simulink library "planetary_gear_lib"  (R2025a)
settings: Solver=VariableStepAuto  StartTime=0.0  StopTime=10.0  RelTol=1e-3
undefined symbols (not defined in the file): cvtPar, Local, rad_planet, rad_sun, X, Y, Z
libraries: sm_lib x24, Multibody_Parts_Lib x15, nesl_utility x2
Description:
  | Copyright 2023-2025 The MathWorks, Inc.
settings Model: Creator=smiller  LastModifiedBy=smiller
settings RTWCC: GPUComputeCapability=3.5

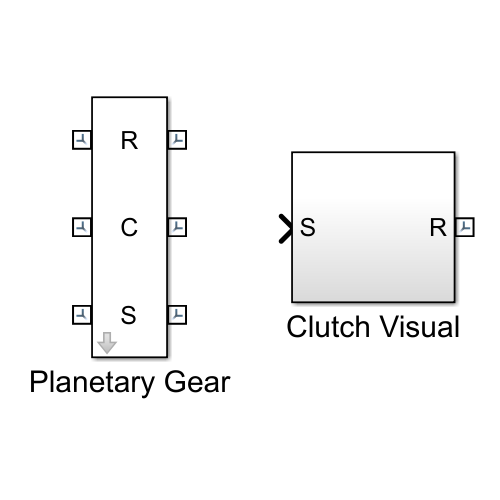
[thumbnail: Simulink's stored preview of the top-level diagram]
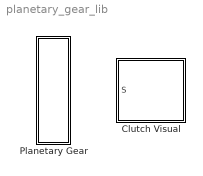
== system planetary_gear_lib ==
  Clutch Visual : Subsystem
  Planetary Gear : Subsystem  Tag=PublishSubsystem  mask{rad_sun=0.78, nteeth_sun=45, rad_planet=0.26, nteeth_planet=15, rad_ring=2*rad_planet+rad_sun, nteeth_ring=75, pg_axial_offset=2, gear_thickness=cvtPar.gear_thickness, link_thickness=cvtPar.link_thickness, rad_hole=cvtPar.rad_hole, ring_gear_clr=[0.0 0.4 0.6], sun_gear_clr=[0.8 0.8 0.3], pla_gear_clr=[0.8 0.8 0.8], carrier_color=[0.5 0.5 0.5]}
      mask prompts: rad_sun "Sun Pitch Radius"; nteeth_sun "Sun # Teeth"; rad_planet "Planet Pitch Radius"; nteeth_planet "Planet # Teeth"; rad_ring "Ring Pitch Radius"; nteeth_ring "Ring # Teeth"; pg_axial_offset "Offset to Planetary Gear (m)"; gear_thickness "Gear Thickness (m)"; link_thickness "Link Thickness (m)"; rad_hole "Gear Hole Radius (m)"; ring_gear_clr "Ring Gear Color [RGB]"; sun_gear_clr "Sun Gear Color [RGB]"; pla_gear_clr "Planet Gear Color [RGB]"; carrier_color "Carrier Color [RGB]"
      mask TypeOptions ring_gear_clr:
      | Ring
      | Gear/gear_clr
      mask TypeOptions sun_gear_clr:
      | Sun
      | Gear/gear_clr
      mask TypeOptions pla_gear_clr: Planet 1/gear_clr | Planet 2/gear_clr | Planet 3/gear_clr
      mask TypeOptions carrier_color:
      | Carrier
      | Gear/carrier_color

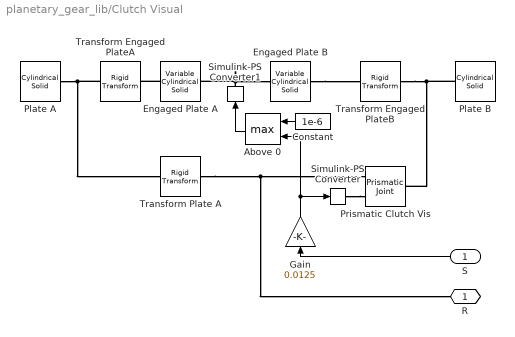
== system planetary_gear_lib/Clutch Visual ==
  S : Inport
  Above 0 : MinMax  Function=max  Inputs=2  ZeroCross=off
  Constant : Constant  Value=1e-6
  Engaged Plate A : sm_lib/Body Elements/Variable Mass/Variable Cylindrical Solid  RadiusType=Constant  Radius=0.025*2+0.001  RadiusUnits=m  LengthType=ProvidedByInput  Length=1  LengthUnits=m  MassType=CalculateFromGeometry  Density=1  DensityUnits=kg/m^3  SenseRadius=off  SenseLength=off  SenseMass=off  SenseCenterOfMass=off  SenseInertiaMatrix=off  GraphicType=FromGeometry  MarkerShape=Sphere  MarkerSize=10  GraphicVisPropType=SimpleVisualProperties  GraphicDiffuseColor=[0.902 0.4784 0.4784]  GraphicOpacity=1.0  GraphicSpecularColor=[0.5 0.5 0.5 1.0]  GraphicAmbientColor=[0.15 0.15 0.15 1.0]  GraphicEmissiveColor=[0.0 0.0 0.0 1.0]  GraphicShininess=75
  Engaged Plate B : sm_lib/Body Elements/Variable Mass/Variable Cylindrical Solid  RadiusType=Constant  Radius=0.025*2+0.001  RadiusUnits=m  LengthType=ProvidedByInput  Length=1  LengthUnits=m  MassType=CalculateFromGeometry  Density=1  DensityUnits=kg/m^3  SenseRadius=off  SenseLength=off  SenseMass=off  SenseCenterOfMass=off  SenseInertiaMatrix=off  GraphicType=FromGeometry  MarkerShape=Sphere  MarkerSize=10  GraphicVisPropType=SimpleVisualProperties  GraphicDiffuseColor=[1 0 0]  GraphicOpacity=1.0  GraphicSpecularColor=[0.5 0.5 0.5 1.0]  GraphicAmbientColor=[0.15 0.15 0.15 1.0]  GraphicEmissiveColor=[0.0 0.0 0.0 1.0]  GraphicShininess=75
  Gain : Gain  Gain=0.0125
  Plate A : sm_lib/Body Elements/Cylindrical Solid  CylinderRadius=0.025*2  CylinderRadiusUnits=m  CylinderLength=0.0125-0.0001  CylinderLengthUnits=m  ExportEntireGeometry=off  InertiaType=CalculateFromGeometry  BasedOnType=Density  Density=1000  DensityUnits=kg/m^3  Mass=1  MassUnits=kg  CenterOfMass=[0 0 0]  CenterOfMassUnits=m  MomentsOfInertia=[1 1 1]  MomentsOfInertiaUnits=kg*m^2  ProductsOfInertia=[0 0 0]  ProductsOfInertiaUnits=kg*m^2  GraphicType=FromGeometry  MarkerShape=Sphere  MarkerSize=10  GraphicVisPropType=SimpleVisualProperties  GraphicDiffuseColor=[1.0 1.0 1.0]  GraphicOpacity=1.0  GraphicSpecularColor=[0.5 0.5 0.5 1.0]  GraphicAmbientColor=[0.15 0.15 0.15 1.0]  GraphicEmissiveColor=[0.0 0.0 0.0 1.0]  GraphicShininess=75  DoExposeReferenceFrame=off  SerializedFrames=<Frames><Frame><Id>Frame1</Id><Value><Name>B</Name><Origin><Source>GeometricFeature</Source><FeatureName>bottom surface</FeatureName></Origin><PrimaryAxis><DefinedDirection>+Z</DefinedDirection><Source>ReferenceFrame</Source><SourceDirection>+Z</SourceDirection><FeatureName></FeatureName></PrimaryAxis><SecondaryAxis><DefinedDirection>+X</DefinedDirection><Source>ReferenceFrame</Source><SourceDirection>+X</SourceDirection><FeatureName></FeatureName></SecondaryAxis></Value></Frame></Frames>
  Plate B : sm_lib/Body Elements/Cylindrical Solid  CylinderRadius=0.025*2  CylinderRadiusUnits=m  CylinderLength=0.0125-0.0001  CylinderLengthUnits=m  ExportEntireGeometry=off  InertiaType=CalculateFromGeometry  BasedOnType=Density  Density=1000  DensityUnits=kg/m^3  Mass=1  MassUnits=kg  CenterOfMass=[0 0 0]  CenterOfMassUnits=m  MomentsOfInertia=[1 1 1]  MomentsOfInertiaUnits=kg*m^2  ProductsOfInertia=[0 0 0]  ProductsOfInertiaUnits=kg*m^2  GraphicType=FromGeometry  MarkerShape=Sphere  MarkerSize=10  GraphicVisPropType=SimpleVisualProperties  GraphicDiffuseColor=[1.0 1.0 1.0]  GraphicOpacity=1.0  GraphicSpecularColor=[0.5 0.5 0.5 1.0]  GraphicAmbientColor=[0.15 0.15 0.15 1.0]  GraphicEmissiveColor=[0.0 0.0 0.0 1.0]  GraphicShininess=75  DoExposeReferenceFrame=off  SerializedFrames=<Frames><Frame><Id>Frame1</Id><Value><Name>F</Name><Origin><Source>GeometricFeature</Source><FeatureName>top surface</FeatureName></Origin><PrimaryAxis><DefinedDirection>+Z</DefinedDirection><Source>ReferenceFrame</Source><SourceDirection>+Z</SourceDirection><FeatureName></FeatureName></PrimaryAxis><SecondaryAxis><DefinedDirection>+X</DefinedDirection><Source>ReferenceFrame</Source><SourceDirection>+X</SourceDirection><FeatureName></FeatureName></SecondaryAxis></Value></Frame></Frames>
  Prismatic Clutch Vis : sm_lib/Joints/Prismatic Joint  JointMode=Normal  CompositeWrenchDir=FollowerOnBase  CompositeWrenchFrame=BaseFrame  SenseConstraintForce=off  SenseConstraintTorque=off  SenseTotalForce=off  SenseTotalTorque=off  PositionTargetSpecify=off  PositionTargetPriority=High  PositionTargetValue=0  PositionTargetValueUnits=m  VelocityTargetSpecify=off  VelocityTargetPriority=High  VelocityTargetValue=0  VelocityTargetValueUnits=m/s  EquilibriumPosition=0  EquilibriumPositionUnits=m  SpringStiffness=0  SpringStiffnessUnits=N/m  DampingCoefficient=0  DampingCoefficientUnits=N/(m/s)  LowerLimitSpecify=off  LowerLimitBound=-1  LowerLimitBoundUnits=m  LowerLimitStiffness=1e6  LowerLimitStiffnessUnits=N/m  LowerLimitDamping=1e3  LowerLimitDampingUnits=N/(m/s)  LowerLimitTransitionRegionWidth=1e-4  LowerLimitTransitionRegionWidthUnits=m  UpperLimitSpecify=off  UpperLimitBound=1  UpperLimitBoundUnits=m  UpperLimitStiffness=1e6  UpperLimitStiffnessUnits=N/m  UpperLimitDamping=1e3  UpperLimitDampingUnits=N/(m/s)  UpperLimitTransitionRegionWidth=1e-4  UpperLimitTransitionRegionWidthUnits=m  TorqueActuationMode=ComputedTorque  MotionActuationMode=InputMotion  SensePosition=off  SenseVelocity=off  SenseAcceleration=off  SenseTorqueForce=off  SenseLowerLimitTorqueForce=off  SenseUpperLimitTorqueForce=off
  Simulink-PS Converter : nesl_utility/Simulink-PS Converter  PhysicalDomain=network_engine_domain  SubClassName=ps_input  LeftPortType=input  RightPortType=output  PseudoPeriodic=off  Frequencies=[]  NoiseDistribution=none  NoiseParameters=[]  Unit=1  AffineConversion=off  FilteringAndDerivatives=filter  SimscapeFilterOrder=2  InputFilterTimeConstant=0.001  UdotUserProvided=0
  Simulink-PS Converter1 : nesl_utility/Simulink-PS Converter  PhysicalDomain=network_engine_domain  SubClassName=ps_input  LeftPortType=input  RightPortType=output  PseudoPeriodic=off  Frequencies=[]  NoiseDistribution=none  NoiseParameters=[]  Unit=1  AffineConversion=off  FilteringAndDerivatives=filter  SimscapeFilterOrder=2  InputFilterTimeConstant=0.001  UdotUserProvided=0
  Transform Engaged PlateA : sm_lib/Frames and Transforms/Rigid Transform  RotationMethod=None  FollAlignAxisA=+X  BaseAlignAxisA=+Y  FollAlignAxisB=+Y  BaseAlignAxisB=+Z  RotationStandardAxis=+Z  RotationAngle=0.0  RotationAngleUnits=deg  RotationArbitraryAxis=[0 0 1]  RotationSequenceAxes=FollowerAxes  RotationSequence=XYX  RotationSequenceAngles=[0 0 0]  RotationSequenceAnglesUnits=deg  RotationMatrix=[1 0 0; 0 1 0; 0 0 1]  Quaternion=[1 0 0 0]  TranslationMethod=StandardAxis  TranslationCartesianOffset=[0 0 0]  TranslationCartesianOffsetUnits=m  TranslationStandardAxis=+Z  TranslationStandardOffset=1e-5  TranslationStandardOffsetUnits=m  TranslationROffset=0  TranslationROffsetUnits=m  TranslationThetaOffset=0  TranslationThetaOffsetUnits=deg  TranslationZOffset=0  TranslationZOffsetUnits=m
  Transform Engaged PlateB : sm_lib/Frames and Transforms/Rigid Transform  RotationMethod=StandardAxis  FollAlignAxisA=+X  BaseAlignAxisA=+Y  FollAlignAxisB=+Y  BaseAlignAxisB=+Z  RotationStandardAxis=+X  RotationAngle=180  RotationAngleUnits=deg  RotationArbitraryAxis=[0 0 1]  RotationSequenceAxes=FollowerAxes  RotationSequence=XYX  RotationSequenceAngles=[0 0 0]  RotationSequenceAnglesUnits=deg  RotationMatrix=[1 0 0; 0 1 0; 0 0 1]  Quaternion=[1 0 0 0]  TranslationMethod=StandardAxis  TranslationCartesianOffset=[0 0 0]  TranslationCartesianOffsetUnits=m  TranslationStandardAxis=+Z  TranslationStandardOffset=-1e-5  TranslationStandardOffsetUnits=m  TranslationROffset=0  TranslationROffsetUnits=m  TranslationThetaOffset=0  TranslationThetaOffsetUnits=deg  TranslationZOffset=0  TranslationZOffsetUnits=m
  Transform Plate A : sm_lib/Frames and Transforms/Rigid Transform  RotationMethod=None  FollAlignAxisA=+X  BaseAlignAxisA=+Y  FollAlignAxisB=+Y  BaseAlignAxisB=+Z  RotationStandardAxis=+Z  RotationAngle=0.0  RotationAngleUnits=deg  RotationArbitraryAxis=[0 0 1]  RotationSequenceAxes=FollowerAxes  RotationSequence=XYX  RotationSequenceAngles=[0 0 0]  RotationSequenceAnglesUnits=deg  RotationMatrix=[1 0 0; 0 1 0; 0 0 1]  Quaternion=[1 0 0 0]  TranslationMethod=StandardAxis  TranslationCartesianOffset=[0 0 0]  TranslationCartesianOffsetUnits=m  TranslationStandardAxis=+Z  TranslationStandardOffset=0.0125  TranslationStandardOffsetUnits=m  TranslationROffset=0  TranslationROffsetUnits=m  TranslationThetaOffset=0  TranslationThetaOffsetUnits=deg  TranslationZOffset=0  TranslationZOffsetUnits=m
  R : PMIOPort  Side=Right
  wires:
  Above 0/1 -> Simulink-PS Converter1/1
  Gain/1 -> Simulink-PS Converter/1, Above 0/2
  Constant/1 -> Above 0/1
  S/1 -> Gain/1
  connections:
  Transform Plate A/LConn1 -- Prismatic Clutch Vis/LConn1 -- R/RConn1
  Engaged Plate B/RConn1 -- Transform Engaged PlateB/LConn1
  Simulink-PS Converter1/RConn1 -- Engaged Plate A/LConn1 -- Engaged Plate B/LConn1
  Plate A/LConn1 -- Transform Engaged PlateA/LConn1 -- Transform Plate A/RConn1
  Transform Engaged PlateB/RConn1 -- Plate B/LConn1 -- Prismatic Clutch Vis/RConn1
  Simulink-PS Converter/RConn1 -- Prismatic Clutch Vis/LConn2
  Engaged Plate A/RConn1 -- Transform Engaged PlateA/RConn1

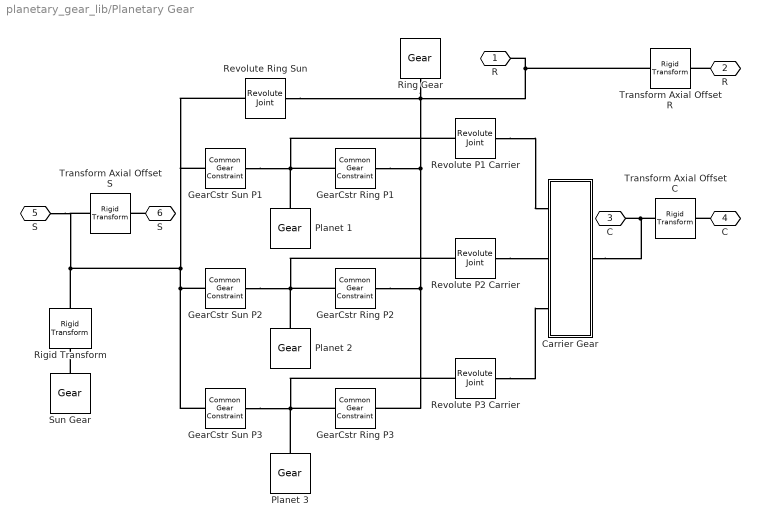
== system planetary_gear_lib/Planetary Gear ==
  Carrier Gear : Subsystem  Tag=PublishSubsystem  mask{carrier_color=carrier_color}
      mask prompts: carrier_color "Carrier Color [RGB]"
      mask TypeOptions carrier_color: Link End P1/circ_color | Link End P2/circ_color | Link End P3/circ_color | Link Seg P1/link_color | Link Seg P2/link_color | Link Seg P3/link_color | Rod P1/rod_color | Rod P2/rod_color | Rod P3/rod_color | Rod Sun/rod_color
  GearCstr Sun P1 : sm_lib/Gears and Couplings/Gears/Common Gear Constraint  GearType=External  SpecificationType=PitchCircleRadii  CenterDistance=20.0  CenterDistanceUnits=cm  GearRatio=1.0  BaseGearRadius=rad_sun  BaseGearRadiusUnits=m  FollGearRadius=rad_planet  FollGearRadiusUnits=m
  GearCstr Sun P2 : sm_lib/Gears and Couplings/Gears/Common Gear Constraint  GearType=External  SpecificationType=PitchCircleRadii  CenterDistance=20.0  CenterDistanceUnits=cm  GearRatio=1.0  BaseGearRadius=rad_sun  BaseGearRadiusUnits=m  FollGearRadius=rad_planet  FollGearRadiusUnits=m
  GearCstr Sun P3 : sm_lib/Gears and Couplings/Gears/Common Gear Constraint  GearType=External  SpecificationType=PitchCircleRadii  CenterDistance=20.0  CenterDistanceUnits=cm  GearRatio=1.0  BaseGearRadius=rad_sun  BaseGearRadiusUnits=m  FollGearRadius=rad_planet  FollGearRadiusUnits=m
  GearCstr Ring P1 : sm_lib/Gears and Couplings/Gears/Common Gear Constraint  GearType=Internal  SpecificationType=PitchCircleRadii  CenterDistance=20.0  CenterDistanceUnits=cm  GearRatio=1.0  BaseGearRadius=rad_ring  BaseGearRadiusUnits=m  FollGearRadius=rad_planet  FollGearRadiusUnits=m
  GearCstr Ring P2 : sm_lib/Gears and Couplings/Gears/Common Gear Constraint  GearType=Internal  SpecificationType=PitchCircleRadii  CenterDistance=20.0  CenterDistanceUnits=cm  GearRatio=1.0  BaseGearRadius=rad_ring  BaseGearRadiusUnits=m  FollGearRadius=rad_planet  FollGearRadiusUnits=m
  GearCstr Ring P3 : sm_lib/Gears and Couplings/Gears/Common Gear Constraint  GearType=Internal  SpecificationType=PitchCircleRadii  CenterDistance=20.0  CenterDistanceUnits=cm  GearRatio=1.0  BaseGearRadius=rad_ring  BaseGearRadiusUnits=m  FollGearRadius=rad_planet  FollGearRadiusUnits=m
  Planet 1 : Multibody_Parts_Lib/Gears/Gear  popup_gear_type=External  gear_pd=rad_planet*2  gear_nt=nteeth_planet  gear_th=gear_thickness  gear_rh=rad_hole  gear_rt=0.02  gear_rho=7000  gear_clr=pla_gear_clr  gear_opc=1  popup_ad_dd=Default  gear_ad=0.125/12  gear_dd=1.157*0.125/12  popup_markings=Two  mark_radius_range=[0.6 0.7]  mark_angle_range=60  mark_color=[1 1 1]*0.2
  Planet 2 : Multibody_Parts_Lib/Gears/Gear  popup_gear_type=External  gear_pd=rad_planet*2  gear_nt=nteeth_planet  gear_th=gear_thickness  gear_rh=rad_hole  gear_rt=0.02  gear_rho=7000  gear_clr=pla_gear_clr  gear_opc=1  popup_ad_dd=Default  gear_ad=0.125/12  gear_dd=1.157*0.125/12  popup_markings=Two  mark_radius_range=[0.6 0.7]  mark_angle_range=60  mark_color=[1 1 1]*0.2
  Planet 3 : Multibody_Parts_Lib/Gears/Gear  popup_gear_type=External  gear_pd=rad_planet*2  gear_nt=nteeth_planet  gear_th=gear_thickness  gear_rh=rad_hole  gear_rt=0.02  gear_rho=7000  gear_clr=pla_gear_clr  gear_opc=1  popup_ad_dd=Default  gear_ad=0.125/12  gear_dd=1.157*0.125/12  popup_markings=Two  mark_radius_range=[0.6 0.7]  mark_angle_range=60  mark_color=[1 1 1]*0.2
  Revolute P1 Carrier : sm_lib/Joints/Revolute Joint  JointMode=Normal  CompositeWrenchDir=FollowerOnBase  CompositeWrenchFrame=BaseFrame  SenseConstraintForce=off  SenseConstraintTorque=off  SenseTotalForce=off  SenseTotalTorque=off  PositionTargetSpecify=off  PositionTargetPriority=High  PositionTargetValue=0  PositionTargetValueUnits=deg  VelocityTargetSpecify=off  VelocityTargetPriority=High  VelocityTargetValue=0  VelocityTargetValueUnits=deg/s  EquilibriumPosition=0  EquilibriumPositionUnits=deg  SpringStiffness=0  SpringStiffnessUnits=N*m/deg  DampingCoefficient=0  DampingCoefficientUnits=N*m/(deg/s)  LowerLimitSpecify=off  LowerLimitBound=-90  LowerLimitBoundUnits=deg  LowerLimitStiffness=1e4  LowerLimitStiffnessUnits=N*m/deg  LowerLimitDamping=10  LowerLimitDampingUnits=N*m/(deg/s)  LowerLimitTransitionRegionWidth=0.1  LowerLimitTransitionRegionWidthUnits=deg  UpperLimitSpecify=off  UpperLimitBound=90  UpperLimitBoundUnits=deg  UpperLimitStiffness=1e4  UpperLimitStiffnessUnits=N*m/deg  UpperLimitDamping=10  UpperLimitDampingUnits=N*m/(deg/s)  UpperLimitTransitionRegionWidth=0.1  UpperLimitTransitionRegionWidthUnits=deg  TorqueActuationMode=NoTorque  MotionActuationMode=ComputedMotion  SensePosition=off  SenseVelocity=off  SenseAcceleration=off  SenseTorqueForce=off  SenseLowerLimitTorqueForce=off  SenseUpperLimitTorqueForce=off
  Revolute P2 Carrier : sm_lib/Joints/Revolute Joint  JointMode=Normal  CompositeWrenchDir=FollowerOnBase  CompositeWrenchFrame=BaseFrame  SenseConstraintForce=off  SenseConstraintTorque=off  SenseTotalForce=off  SenseTotalTorque=off  PositionTargetSpecify=off  PositionTargetPriority=High  PositionTargetValue=0  PositionTargetValueUnits=deg  VelocityTargetSpecify=off  VelocityTargetPriority=High  VelocityTargetValue=0  VelocityTargetValueUnits=deg/s  EquilibriumPosition=0  EquilibriumPositionUnits=deg  SpringStiffness=0  SpringStiffnessUnits=N*m/deg  DampingCoefficient=0  DampingCoefficientUnits=N*m/(deg/s)  LowerLimitSpecify=off  LowerLimitBound=-90  LowerLimitBoundUnits=deg  LowerLimitStiffness=1e4  LowerLimitStiffnessUnits=N*m/deg  LowerLimitDamping=10  LowerLimitDampingUnits=N*m/(deg/s)  LowerLimitTransitionRegionWidth=0.1  LowerLimitTransitionRegionWidthUnits=deg  UpperLimitSpecify=off  UpperLimitBound=90  UpperLimitBoundUnits=deg  UpperLimitStiffness=1e4  UpperLimitStiffnessUnits=N*m/deg  UpperLimitDamping=10  UpperLimitDampingUnits=N*m/(deg/s)  UpperLimitTransitionRegionWidth=0.1  UpperLimitTransitionRegionWidthUnits=deg  TorqueActuationMode=NoTorque  MotionActuationMode=ComputedMotion  SensePosition=off  SenseVelocity=off  SenseAcceleration=off  SenseTorqueForce=off  SenseLowerLimitTorqueForce=off  SenseUpperLimitTorqueForce=off
  Revolute P3 Carrier : sm_lib/Joints/Revolute Joint  JointMode=Normal  CompositeWrenchDir=FollowerOnBase  CompositeWrenchFrame=BaseFrame  SenseConstraintForce=off  SenseConstraintTorque=off  SenseTotalForce=off  SenseTotalTorque=off  PositionTargetSpecify=off  PositionTargetPriority=High  PositionTargetValue=0  PositionTargetValueUnits=deg  VelocityTargetSpecify=off  VelocityTargetPriority=High  VelocityTargetValue=0  VelocityTargetValueUnits=deg/s  EquilibriumPosition=0  EquilibriumPositionUnits=deg  SpringStiffness=0  SpringStiffnessUnits=N*m/deg  DampingCoefficient=0  DampingCoefficientUnits=N*m/(deg/s)  LowerLimitSpecify=off  LowerLimitBound=-90  LowerLimitBoundUnits=deg  LowerLimitStiffness=1e4  LowerLimitStiffnessUnits=N*m/deg  LowerLimitDamping=10  LowerLimitDampingUnits=N*m/(deg/s)  LowerLimitTransitionRegionWidth=0.1  LowerLimitTransitionRegionWidthUnits=deg  UpperLimitSpecify=off  UpperLimitBound=90  UpperLimitBoundUnits=deg  UpperLimitStiffness=1e4  UpperLimitStiffnessUnits=N*m/deg  UpperLimitDamping=10  UpperLimitDampingUnits=N*m/(deg/s)  UpperLimitTransitionRegionWidth=0.1  UpperLimitTransitionRegionWidthUnits=deg  TorqueActuationMode=NoTorque  MotionActuationMode=ComputedMotion  SensePosition=off  SenseVelocity=off  SenseAcceleration=off  SenseTorqueForce=off  SenseLowerLimitTorqueForce=off  SenseUpperLimitTorqueForce=off
  Revolute Ring Sun : sm_lib/Joints/Revolute Joint  JointMode=Normal  CompositeWrenchDir=FollowerOnBase  CompositeWrenchFrame=BaseFrame  SenseConstraintForce=off  SenseConstraintTorque=off  SenseTotalForce=off  SenseTotalTorque=off  PositionTargetSpecify=off  PositionTargetPriority=High  PositionTargetValue=0  PositionTargetValueUnits=deg  VelocityTargetSpecify=off  VelocityTargetPriority=High  VelocityTargetValue=0  VelocityTargetValueUnits=deg/s  EquilibriumPosition=0  EquilibriumPositionUnits=deg  SpringStiffness=0  SpringStiffnessUnits=N*m/deg  DampingCoefficient=0  DampingCoefficientUnits=N*m/(deg/s)  LowerLimitSpecify=off  LowerLimitBound=-90  LowerLimitBoundUnits=deg  LowerLimitStiffness=1e4  LowerLimitStiffnessUnits=N*m/deg  LowerLimitDamping=10  LowerLimitDampingUnits=N*m/(deg/s)  LowerLimitTransitionRegionWidth=0.1  LowerLimitTransitionRegionWidthUnits=deg  UpperLimitSpecify=off  UpperLimitBound=90  UpperLimitBoundUnits=deg  UpperLimitStiffness=1e4  UpperLimitStiffnessUnits=N*m/deg  UpperLimitDamping=10  UpperLimitDampingUnits=N*m/(deg/s)  UpperLimitTransitionRegionWidth=0.1  UpperLimitTransitionRegionWidthUnits=deg  TorqueActuationMode=NoTorque  MotionActuationMode=ComputedMotion  SensePosition=off  SenseVelocity=off  SenseAcceleration=off  SenseTorqueForce=off  SenseLowerLimitTorqueForce=off  SenseUpperLimitTorqueForce=off
  Rigid Transform : sm_lib/Frames and Transforms/Rigid Transform  RotationMethod=StandardAxis  FollAlignAxisA=+X  BaseAlignAxisA=+Y  FollAlignAxisB=+Y  BaseAlignAxisB=+Z  RotationStandardAxis=+Z  RotationAngle=360/nteeth_sun/2  RotationAngleUnits=deg  RotationArbitraryAxis=[0 0 1]  RotationSequenceAxes=FollowerAxes  RotationSequence=XYX  RotationSequenceAngles=[0 0 0]  RotationSequenceAnglesUnits=deg  RotationMatrix=[1 0 0; 0 1 0; 0 0 1]  Quaternion=[1 0 0 0]  TranslationMethod=None  TranslationCartesianOffset=[0 0 0]  TranslationCartesianOffsetUnits=m  TranslationStandardAxis=+Z  TranslationStandardOffset=0  TranslationStandardOffsetUnits=m  TranslationROffset=0  TranslationROffsetUnits=m  TranslationThetaOffset=0  TranslationThetaOffsetUnits=deg  TranslationZOffset=0  TranslationZOffsetUnits=m
  Ring Gear : Multibody_Parts_Lib/Gears/Gear  popup_gear_type=Internal  gear_pd=rad_ring*2  gear_nt=nteeth_ring  gear_th=gear_thickness  gear_rh=0.05  gear_rt=rad_ring*0.1  gear_rho=7000  gear_clr=ring_gear_clr  gear_opc=1  popup_ad_dd=Default  gear_ad=0.125/12  gear_dd=1.157*0.125/12  popup_markings=Two  mark_radius_range=[1.06 1.1]  mark_angle_range=60  mark_color=[1 1 1]
  Sun Gear : Multibody_Parts_Lib/Gears/Gear  popup_gear_type=External  gear_pd=rad_sun*2  gear_nt=nteeth_sun  gear_th=gear_thickness  gear_rh=rad_hole  gear_rt=0.02  gear_rho=7000  gear_clr=sun_gear_clr  gear_opc=1  popup_ad_dd=Default  gear_ad=0.125/12  gear_dd=1.157*0.125/12  popup_markings=Two  mark_radius_range=[0.6 0.7]  mark_angle_range=60  mark_color=[1 1 1]*0.2
  Transform Axial Offset C : sm_lib/Frames and Transforms/Rigid Transform  RotationMethod=None  FollAlignAxisA=+X  BaseAlignAxisA=+Y  FollAlignAxisB=+Y  BaseAlignAxisB=+Z  RotationStandardAxis=+Z  RotationAngle=0.0  RotationAngleUnits=deg  RotationArbitraryAxis=[0 0 1]  RotationSequenceAxes=FollowerAxes  RotationSequence=XYX  RotationSequenceAngles=[0 0 0]  RotationSequenceAnglesUnits=deg  RotationMatrix=[1 0 0; 0 1 0; 0 0 1]  Quaternion=[1 0 0 0]  TranslationMethod=StandardAxis  TranslationCartesianOffset=[0 0 0]  TranslationCartesianOffsetUnits=m  TranslationStandardAxis=+Z  TranslationStandardOffset=pg_axial_offset  TranslationStandardOffsetUnits=m  TranslationROffset=0  TranslationROffsetUnits=m  TranslationThetaOffset=0  TranslationThetaOffsetUnits=deg  TranslationZOffset=0  TranslationZOffsetUnits=m
  Transform Axial Offset R : sm_lib/Frames and Transforms/Rigid Transform  RotationMethod=None  FollAlignAxisA=+X  BaseAlignAxisA=+Y  FollAlignAxisB=+Y  BaseAlignAxisB=+Z  RotationStandardAxis=+Z  RotationAngle=0.0  RotationAngleUnits=deg  RotationArbitraryAxis=[0 0 1]  RotationSequenceAxes=FollowerAxes  RotationSequence=XYX  RotationSequenceAngles=[0 0 0]  RotationSequenceAnglesUnits=deg  RotationMatrix=[1 0 0; 0 1 0; 0 0 1]  Quaternion=[1 0 0 0]  TranslationMethod=StandardAxis  TranslationCartesianOffset=[0 0 0]  TranslationCartesianOffsetUnits=m  TranslationStandardAxis=+Z  TranslationStandardOffset=pg_axial_offset  TranslationStandardOffsetUnits=m  TranslationROffset=0  TranslationROffsetUnits=m  TranslationThetaOffset=0  TranslationThetaOffsetUnits=deg  TranslationZOffset=0  TranslationZOffsetUnits=m
  Transform Axial Offset S : sm_lib/Frames and Transforms/Rigid Transform  RotationMethod=None  FollAlignAxisA=+X  BaseAlignAxisA=+Y  FollAlignAxisB=+Y  BaseAlignAxisB=+Z  RotationStandardAxis=+Z  RotationAngle=0.0  RotationAngleUnits=deg  RotationArbitraryAxis=[0 0 1]  RotationSequenceAxes=FollowerAxes  RotationSequence=XYX  RotationSequenceAngles=[0 0 0]  RotationSequenceAnglesUnits=deg  RotationMatrix=[1 0 0; 0 1 0; 0 0 1]  Quaternion=[1 0 0 0]  TranslationMethod=StandardAxis  TranslationCartesianOffset=[0 0 0]  TranslationCartesianOffsetUnits=m  TranslationStandardAxis=+Z  TranslationStandardOffset=pg_axial_offset  TranslationStandardOffsetUnits=m  TranslationROffset=0  TranslationROffsetUnits=m  TranslationThetaOffset=0  TranslationThetaOffsetUnits=deg  TranslationZOffset=0  TranslationZOffsetUnits=m
  "   R" : PMIOPort  Side=Left
  R : PMIOPort  Port=2  Side=Right
  "   C" : PMIOPort  Port=3  Side=Left
  C : PMIOPort  Port=4  Side=Right
  "   S" : PMIOPort  Port=5  Side=Left
  S : PMIOPort  Port=6  Side=Right
  connections:
  C/RConn1 -- Transform Axial Offset C/RConn1
  GearCstr Ring P2/RConn1 -- Revolute P2 Carrier/LConn1 -- Planet 2/RConn1 -- GearCstr Sun P2/RConn1
  GearCstr Ring P1/RConn1 -- Revolute P1 Carrier/LConn1 -- Planet 1/RConn1 -- GearCstr Sun P1/RConn1
  GearCstr Ring P3/RConn1 -- Revolute P3 Carrier/LConn1 -- Planet 3/RConn1 -- GearCstr Sun P3/RConn1
  GearCstr Sun P2/LConn1 -- GearCstr Sun P3/LConn1 -- GearCstr Sun P1/LConn1 -- Revolute Ring Sun/RConn1 -- Rigid Transform/LConn1 -- Transform Axial Offset S/LConn1 -- "   S"/RConn1
  Revolute Ring Sun/LConn1 -- "   R"/RConn1 -- Transform Axial Offset R/LConn1 -- Ring Gear/RConn1 -- GearCstr Ring P1/LConn1 -- GearCstr Ring P3/LConn1 -- GearCstr Ring P2/LConn1
  Revolute P1 Carrier/RConn1 -- Carrier Gear/LConn1
  Revolute P2 Carrier/RConn1 -- Carrier Gear/LConn2
  Revolute P3 Carrier/RConn1 -- Carrier Gear/LConn3
  R/RConn1 -- Transform Axial Offset R/RConn1
  Transform Axial Offset C/LConn1 -- Carrier Gear/RConn1 -- "   C"/RConn1
  S/RConn1 -- Transform Axial Offset S/RConn1
  Sun Gear/RConn1 -- Rigid Transform/RConn1

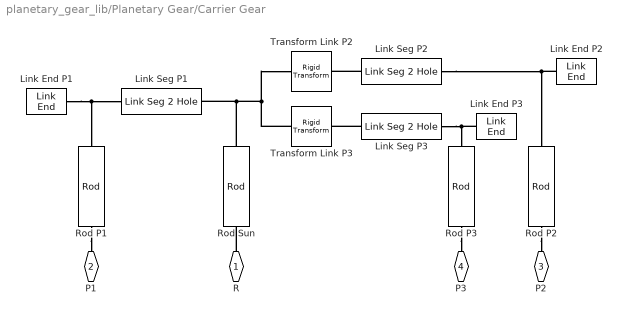
== system planetary_gear_lib/Planetary Gear/Carrier Gear ==
  Link End P1 : Multibody_Parts_Lib/Linkages/Link End  circ_radout=rad_hole*2  circ_radin=rad_hole  popup_holelr=+X  deg_1=-90  deg_2=90  circ_len=link_thickness  circ_rho=7000  circ_color=carrier_color  circ_opc=1
  Link End P2 : Multibody_Parts_Lib/Linkages/Link End  circ_radout=rad_hole*2  circ_radin=rad_hole  popup_holelr=+X  deg_1=-90  deg_2=90  circ_len=link_thickness  circ_rho=7000  circ_color=carrier_color  circ_opc=1
  Link End P3 : Multibody_Parts_Lib/Linkages/Link End  circ_radout=rad_hole*2  circ_radin=rad_hole  popup_holelr=+X  deg_1=-90  deg_2=90  circ_len=link_thickness  circ_rho=7000  circ_color=carrier_color  circ_opc=1
  Link Seg P1 : Multibody_Parts_Lib/Linkages/Link Seg 2 Hole  link_len=rad_sun+rad_planet  link_width=rad_hole*2*2  link_radh=rad_hole  link_thickness=link_thickness  link_rho=7000  link_color=carrier_color  link_opc=1
  Link Seg P2 : Multibody_Parts_Lib/Linkages/Link Seg 2 Hole  link_len=rad_sun+rad_planet  link_width=rad_hole*2*2  link_radh=rad_hole  link_thickness=link_thickness  link_rho=7000  link_color=carrier_color  link_opc=1
  Link Seg P3 : Multibody_Parts_Lib/Linkages/Link Seg 2 Hole  link_len=rad_sun+rad_planet  link_width=rad_hole*2*2  link_radh=rad_hole  link_thickness=link_thickness  link_rho=7000  link_color=carrier_color  link_opc=1
  Rod P1 : Multibody_Parts_Lib/Basic/Rod  rod_rad=rad_hole  rod_len=gear_thickness  rod_rho=7000  rod_color=carrier_color  rod_opc=1  popup_zori=Local +Z  popup_markings=None  mark_radius_range=[0.5 1.01]  mark_length_range=1.005  mark_angle_range=30  mark_color=[1 1 1]
  Rod P2 : Multibody_Parts_Lib/Basic/Rod  rod_rad=rad_hole  rod_len=gear_thickness  rod_rho=7000  rod_color=carrier_color  rod_opc=1  popup_zori=Local +Z  popup_markings=None  mark_radius_range=[0.5 1.01]  mark_length_range=1.005  mark_angle_range=30  mark_color=[1 1 1]
  Rod P3 : Multibody_Parts_Lib/Basic/Rod  rod_rad=rad_hole  rod_len=gear_thickness  rod_rho=7000  rod_color=carrier_color  rod_opc=1  popup_zori=Local +Z  popup_markings=None  mark_radius_range=[0.5 1.01]  mark_length_range=1.005  mark_angle_range=30  mark_color=[1 1 1]
  Rod Sun : Multibody_Parts_Lib/Basic/Rod  rod_rad=rad_hole  rod_len=gear_thickness  rod_rho=7000  rod_color=carrier_color  rod_opc=1*0  popup_zori=Local +Z  popup_markings=None  mark_radius_range=[0.5 1.01]  mark_length_range=1.005  mark_angle_range=30  mark_color=[1 1 1]
  Transform Link P2 : sm_lib/Frames and Transforms/Rigid Transform  RotationMethod=StandardAxis  FollAlignAxisA=+X  BaseAlignAxisA=+Y  FollAlignAxisB=+Y  BaseAlignAxisB=+Z  RotationStandardAxis=+Z  RotationAngle=120  RotationAngleUnits=deg  RotationArbitraryAxis=[0 0 1]  RotationSequenceAxes=FollowerAxes  RotationSequence=XYX  RotationSequenceAngles=[0 0 0]  RotationSequenceAnglesUnits=deg  RotationMatrix=[1 0 0; 0 1 0; 0 0 1]  Quaternion=[1 0 0 0]  TranslationMethod=None  TranslationCartesianOffset=[0 0 0]  TranslationCartesianOffsetUnits=m  TranslationStandardAxis=+Z  TranslationStandardOffset=0  TranslationStandardOffsetUnits=m  TranslationROffset=0  TranslationROffsetUnits=m  TranslationThetaOffset=0  TranslationThetaOffsetUnits=deg  TranslationZOffset=0  TranslationZOffsetUnits=m
  Transform Link P3 : sm_lib/Frames and Transforms/Rigid Transform  RotationMethod=StandardAxis  FollAlignAxisA=+X  BaseAlignAxisA=+Y  FollAlignAxisB=+Y  BaseAlignAxisB=+Z  RotationStandardAxis=+Z  RotationAngle=-120  RotationAngleUnits=deg  RotationArbitraryAxis=[0 0 1]  RotationSequenceAxes=FollowerAxes  RotationSequence=XYX  RotationSequenceAngles=[0 0 0]  RotationSequenceAnglesUnits=deg  RotationMatrix=[1 0 0; 0 1 0; 0 0 1]  Quaternion=[1 0 0 0]  TranslationMethod=None  TranslationCartesianOffset=[0 0 0]  TranslationCartesianOffsetUnits=m  TranslationStandardAxis=+Z  TranslationStandardOffset=0  TranslationStandardOffsetUnits=m  TranslationROffset=0  TranslationROffsetUnits=m  TranslationThetaOffset=0  TranslationThetaOffsetUnits=deg  TranslationZOffset=0  TranslationZOffsetUnits=m
  R : PMIOPort  Side=Right
  P1 : PMIOPort  Port=2  Side=Left
  P2 : PMIOPort  Port=3  Side=Left
  P3 : PMIOPort  Port=4  Side=Left
  connections:
  Rod P1/LConn1 -- P1/RConn1
  Link End P1/LConn1 -- Rod P1/RConn1 -- Link Seg P1/RConn1
  Rod Sun/RConn1 -- Transform Link P3/LConn1 -- Transform Link P2/LConn1 -- Link Seg P1/LConn1
  Link Seg P2/RConn1 -- Link End P2/LConn1 -- Rod P2/RConn1
  Link Seg P2/LConn1 -- Transform Link P2/RConn1
  R/RConn1 -- Rod Sun/LConn1
  Link Seg P3/RConn1 -- Rod P3/RConn1 -- Link End P3/LConn1
  Link Seg P3/LConn1 -- Transform Link P3/RConn1
  Rod P2/LConn1 -- P2/RConn1
  Rod P3/LConn1 -- P3/RConn1
